simulink model "inverted_pendulum"  (R2025b)
settings: Solver=VariableStepAuto  StartTime=0.0  StopTime=30  RelTol=1e-3
settings Model: Creator=ASUS  LastModifiedBy=ASUS

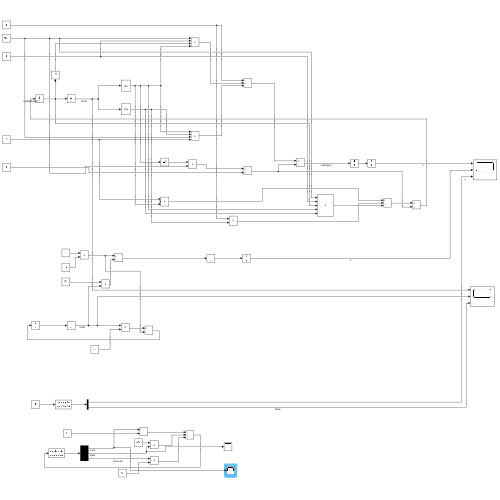
[thumbnail: Simulink's stored preview of the top-level diagram]
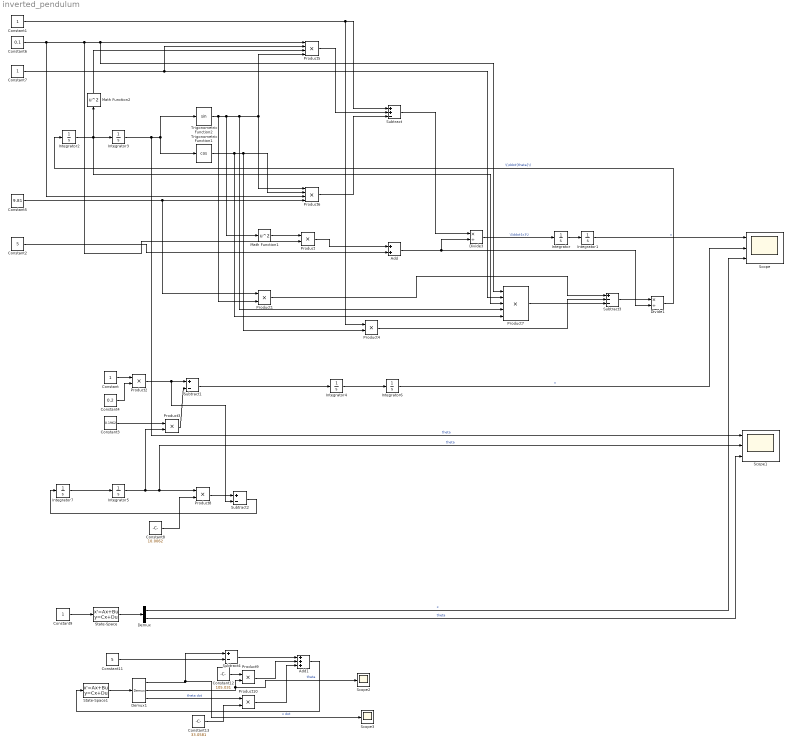
== system inverted_pendulum ==
  Add : Sum
  Add1 : Sum  Inputs=+++
  Constant{,1,7,9} (4 alike) : Constant
  Constant11 : Constant  Value=5
  Constant12 : Constant  Value=105.031
  Constant13 : Constant  Value=33.0581
  Constant2 : Constant  Value=5
  Constant3 : Constant  Value=0.1962
  Constant4 : Constant  Value=0.2
  Constant5 : Constant  Value=9.81
  Constant6 : Constant  Value=0.1
  Constant8 : Constant  Value=10.0062
  Demux : Demux  Outputs=2
  Demux1 : Demux  Outputs=3
  Divide1 : Product  Inputs=*/
  Divide3 : Product  Inputs=*/
  Integrator{,1..2,4,6..7} (6 alike) : Integrator
  Integrator3 : Integrator  InitialCondition=0.01
  Integrator5 : Integrator  InitialCondition=0.01
  Math Function1 : Math  Operator=square
  Math Function2 : Math  Operator=square
  Product{,2..4,8..10} (7 alike) : Product
  Product1 : Product  Inputs=3
  Product5 : Product  Inputs=4
  Product6 : Product  Inputs=4
  Product7 : Product  Inputs=5
  Scope : Scope  NumInputPorts=3
      settings: ActiveDisplayYMinimum=-0.16206004529732521  ActiveDisplayYMaximum=0.55061120351465942
  Scope1 : Scope  NumInputPorts=3
      settings: ActiveDisplayYMinimum=-5.0989771279419909  ActiveDisplayYMaximum=1.4597351396271869
  Scope2 : Scope
      settings: ActiveDisplayYMinimum=-0.0341074794625076  ActiveDisplayYMaximum=0.15331222871857175  DataLoggingVariableName=ScopeData2
  Scope3 : Scope
      settings: ActiveDisplayYMinimum=-2.8896319002987951  ActiveDisplayYMaximum=6.3248183210193591  DataLoggingVariableName=ScopeData3
  State-Space : StateSpace  A=[0 1 0 0; 0 0 -0.1962 0; 0 0 0 1; 0 0 10.0062 0]  B=[0; 0.2; 0; -0.2]  C=[1 0 0 0; 0 0 1 0]  D=[0; 0]  InitialCondition=[0; 0; 0.01; 0]
  State-Space1 : StateSpace  A=[0 1 0 0; 0 0 -0.1962 0; 0 0 0 1; 0 0 10.0062 0]  B=[0; 0.2; 0; -0.2]  C=[0 1 0 0; 0 0 1 0; 0 0 0 1]  D=[0; 0; 0]  InitialCondition=[0; 0; 0.01; 0]
  Subtract : Sum  Inputs=++-
  Subtract1 : Sum  Inputs=+-
  Subtract2 : Sum  Inputs=+-
  Subtract3 : Sum  Inputs=+--
  Subtract4 : Sum  Inputs=+-
  Trigonometric Function1 : Trigonometry  Operator=cos
  Trigonometric Function2 : Trigonometry
  wires:
  Integrator/1 -> Integrator1/1
  Integrator1/1 -> Scope/1  "x"
  Divide3/1 -> Integrator/1  "\\(\\ddot{x}\\)"
  Divide1/1 -> Integrator2/1  "\\(\\ddot{theta}\\)"
  Integrator3/1 -> Scope1/1, Trigonometric Function1/1, Trigonometric Function2/1  "theta"
  Integrator2/1 -> Product7/3, Math Function2/1, Integrator3/1
  Constant6/1 -> Product6/3, Product/2, Product7/1, Product5/1
  Constant7/1 -> Product7/2, Product5/2
  Trigonometric Function2/1 -> Product1/3, Math Function1/1, Product7/4, Product6/1, Product5/4
  Constant5/1 -> Product1/1, Product6/4
  Trigonometric Function1/1 -> Product7/5, Product4/2, Product6/2
  Product5/1 -> Subtract/2
  Product6/1 -> Subtract/3
  Math Function1/1 -> Product/1
  Subtract/1 -> Divide3/1
  Constant1/1 -> Subtract/1, Product4/1
  Product1/1 -> Subtract3/1
  Product4/1 -> Subtract3/2
  Product7/1 -> Subtract3/3
  Subtract3/1 -> Divide1/1
  Subtract1/1 -> Integrator4/1
  Integrator4/1 -> Integrator6/1
  Integrator6/1 -> Scope/2  "x"
  Subtract2/1 -> Integrator7/1
  Integrator7/1 -> Integrator5/1
  Integrator5/1 -> Scope1/2, Product8/1, Product3/2  "theta"
  Constant/1 -> Product2/1
  Constant4/1 -> Product2/2
  Product2/1 -> Subtract2/2, Subtract1/1
  Constant3/1 -> Product3/1
  Product3/1 -> Subtract1/2
  Constant8/1 -> Product8/2
  Product8/1 -> Subtract2/1
  Constant9/1 -> State-Space/1
  State-Space/1 -> Demux/1
  Demux/1 -> Scope/3  "x"
  Demux/2 -> Scope1/3  "theta"
  Add/1 -> Divide3/2, Divide1/2
  Constant2/1 -> Add/2
  Product/1 -> Add/1
  Math Function2/1 -> Product5/3
  Add1/1 -> State-Space1/1
  State-Space1/1 -> Demux1/1
  Demux1/1 -> Scope3/1, Subtract4/1  "x dot"
  Demux1/2 -> Scope2/1, Product9/2  "theta"
  Demux1/3 -> Product10/1  "theta dot"
  Constant11/1 -> Subtract4/2
  Subtract4/1 -> Add1/1
  Constant12/1 -> Product9/1
  Product9/1 -> Add1/2
  Constant13/1 -> Product10/2
  Product10/1 -> Add1/3
